simulink model "ot_security_demo"  (R2026a)
settings: Solver=FixedStepDiscrete  StopTime=2015  FixedStep=1
settings Model: Creator=suraj  LastModifiedBy=suraj

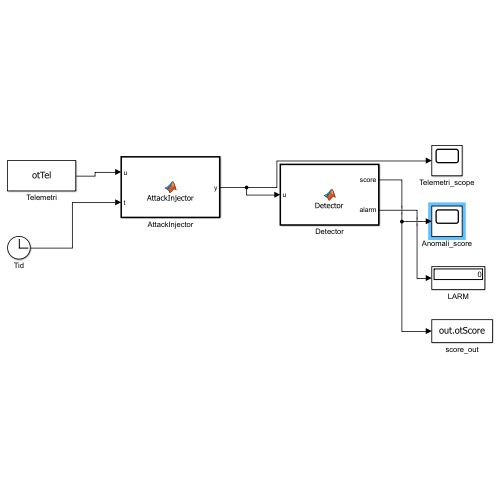
[thumbnail: Simulink's stored preview of the top-level diagram]
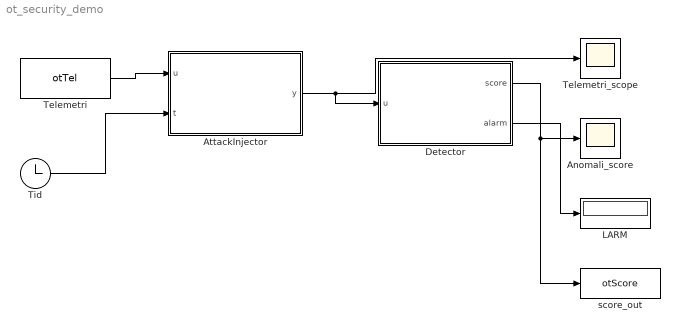
== system ot_security_demo ==
  Anomali_score : Scope
      settings: ActiveDisplayYMinimum=-1423.4586204039251  ActiveDisplayYMaximum=12813.832449931118
  AttackInjector : MATLAB Function  TreatAsAtomicUnit=on
  Detector : MATLAB Function  TreatAsAtomicUnit=on
  LARM : Display
  Telemetri : FromWorkspace  VariableName=otTel  Interpolate=off  OutputAfterFinalValue=Holding final value
  Telemetri_scope : Scope
      settings: ActiveDisplayYMinimum=-95.04996601920358  ActiveDisplayYMaximum=904.00292948718493
  Tid : Clock
  score_out : ToWorkspace  VariableName=otScore  SaveFormat=Timeseries  SampleTime=-1
  wires:
  Telemetri/1 -> AttackInjector/1(u)
  Tid/1 -> AttackInjector/2(t)
  AttackInjector/1(y) -> Detector/1(u), Telemetri_scope/1
  Detector/1(score) -> Anomali_score/1, score_out/1
  Detector/2(alarm) -> LARM/1

== matlab function ot_security_demo/AttackInjector ==
  data: u input; y output; t input
function y = AttackInjector(u, t)
%#codegen
% Live attack injection (simulated effects only)
y = u;
if t>=900 && t<=1000
    y(1) = 88;            % sensor spoofing: forged supply temp
elseif t>=1150 && t<=1200
    y(1) = u(1) + 20;     % command injection: overheating
elseif t>=1780 && t<=1840
    y(4) = 50 + 40*sin(2*pi*t/3);   % ransomware: erratic pump
    y(5) = u(5) + 1.5;              % pressure spike
end
end

== matlab function ot_security_demo/Detector ==
  data: u input; score output; alarm output
function [score, alarm] = Detector(u)
%#codegen
% Online Mahalanobis-distance detector (baseline learned offline)
mu = [85.5172 45.7815 566.947 52.8464 5.41677];
Sinv = [27.4401 -27.201 -0.0712352 -0.0640848 3.55033;-27.201 27.2804 0.0564635 0.0407198 -3.96188;-0.0712352 0.0564635 0.0123529 -0.0559894 -0.90169;-0.0640848 0.0407198 -0.0559894 0.369288 -0.518479;3.55033 -3.96188 -0.90169 -0.518479 396.948];
thr = 19.6035;
dv = u(:).' - mu;
score = dv * Sinv * dv.';
alarm = double(score > thr);
end
